simulink model "IEEE39_Simulink_FMU_Cosim_Validation"  (R2025a)
settings: Solver=ode4  StartTime=0.0  StopTime=stopTime  FixedStep=dt  RelTol=1e-3
values from neighbouring files (symbols this model uses):
  dt = double(entry.step_s)    [run_fmu_cosim_sweep.m]    (also in run_ieee39_closed_loop.m; run_ieee39_native_closed_loop.m)
  i0 = localPassiveCurrent(vabc(1,:))    [run_fmu_cosim_sweep.m]
settings Model: Creator=matthiasmees  LastModifiedBy=matthiasmees
settings DataIOCC: SaveOutput=off  SaveTime=off

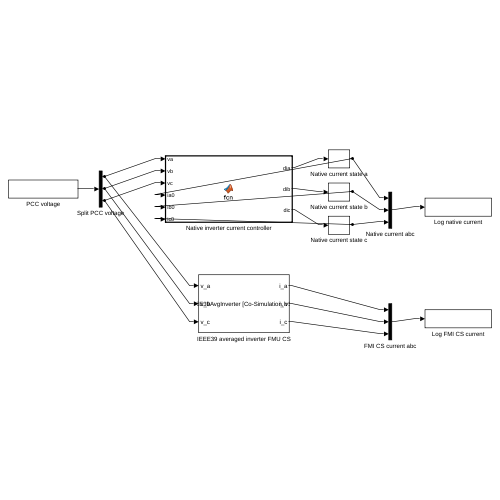
[thumbnail: Simulink's stored preview of the top-level diagram]
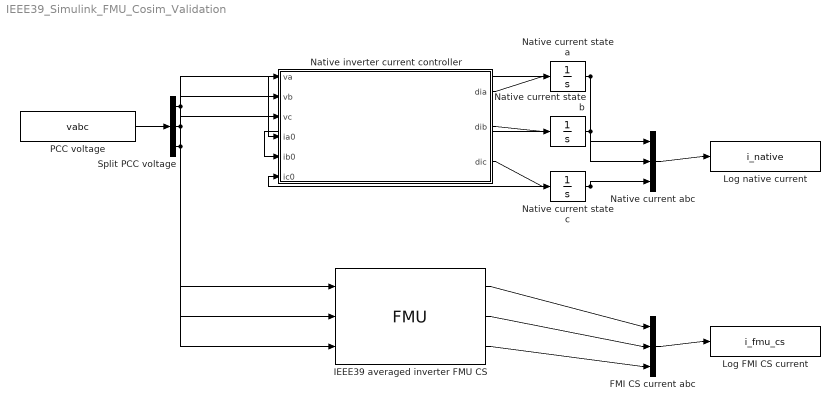
== system IEEE39_Simulink_FMU_Cosim_Validation ==
  FMI CS current abc : Mux  Inputs=3
  IEEE39 averaged inverter FMU CS : FMU  FMUName=IEEE39AvgInverter.fmu  FMUInputMapping=Flat  FMUOutputMapping=Flat  FMUMode=CoSimulation
      mask Type: IEEE39AvgInverter [Co-Simulation, v3.0]
      mask Display:
      | disp('IEEE39AvgInverter [Co-Simulation, v3.0]');
      | port_label('output',1,'i_a');
      | port_label('output',2,'i_b');
      | port_label('output',3,'i_c');
      | port_label('input',1,'v_a');
      | port_label('input',2,'v_b');
      | port_label('input',3,'v_c');
  Log FMI CS current : ToWorkspace  VariableName=i_fmu_cs  SaveFormat=Timeseries  SampleTime=-1
  Log native current : ToWorkspace  VariableName=i_native  SaveFormat=Timeseries  SampleTime=-1
  Native current abc : Mux  Inputs=3
  Native current state a : Integrator  InitialCondition=i0(1)
  Native current state b : Integrator  InitialCondition=i0(2)
  Native current state c : Integrator  InitialCondition=i0(3)
  Native inverter current controller : MATLAB Function  TreatAsAtomicUnit=on
  PCC voltage : FromWorkspace  VariableName=vabc  SampleTime=dt
  Split PCC voltage : Demux  Outputs=3
  wires:
  PCC voltage/1 -> Split PCC voltage/1
  Split PCC voltage/1 -> Native inverter current controller/1(va), IEEE39 averaged inverter FMU CS/1
  Native current state a/1 -> Native inverter current controller/4(ia0), Native current abc/1
  Native inverter current controller/1(dia) -> Native current state a/1
  IEEE39 averaged inverter FMU CS/1 -> FMI CS current abc/1
  Split PCC voltage/2 -> Native inverter current controller/2(vb), IEEE39 averaged inverter FMU CS/2
  Native current state b/1 -> Native inverter current controller/5(ib0), Native current abc/2
  Native inverter current controller/2(dib) -> Native current state b/1
  IEEE39 averaged inverter FMU CS/2 -> FMI CS current abc/2
  Split PCC voltage/3 -> Native inverter current controller/3(vc), IEEE39 averaged inverter FMU CS/3
  Native current state c/1 -> Native inverter current controller/6(ic0), Native current abc/3
  Native inverter current controller/3(dic) -> Native current state c/1
  IEEE39 averaged inverter FMU CS/3 -> FMI CS current abc/3
  Native current abc/1 -> Log native current/1
  FMI CS current abc/1 -> Log FMI CS current/1

== matlab function IEEE39_Simulink_FMU_Cosim_Validation/Native inverter current controller ==
  data: va input; dia output; vb input; vc input; ia0 input; ib0 input; ic0 input; dib output; dic output
function [dia,dib,dic] = fcn(va,vb,vc,ia0,ib0,ic0)
%#codegen
P=125e6; Q=80.881e6; Vnom=345e3; Ipu=1.20; tau=5e-3;
a=(2/3)*(va-0.5*vb-0.5*vc);
b=(2/3)*(sqrt(3)/2)*(vb-vc); v2=a*a+b*b;
if v2<1, iaref=0; ibref=0; icref=0; else
 k=2/(3*v2); ialpha=k*(P*a+Q*b); ibeta=k*(P*b-Q*a);
 imax=Ipu*sqrt(2)*hypot(P,Q)/(sqrt(3)*Vnom); imag=hypot(ialpha,ibeta);
 if imag>imax, ialpha=ialpha*imax/imag; ibeta=ibeta*imax/imag; end
 iaref=ialpha; ibref=-0.5*ialpha+sqrt(3)/2*ibeta;
 icref=-0.5*ialpha-sqrt(3)/2*ibeta; end
 dia=(-iaref-ia0)/tau; dib=(-ibref-ib0)/tau; dic=(-icref-ic0)/tau;
end
